simulink model "KC200GT"  (R2023a)
settings: Solver=ode1  StartTime=0.0  StopTime=1  FixedStep=1e-4  RelTol=1e-3
libraries: simulink x1
settings Model: Creator=Solal  LastModifiedBy=Solal

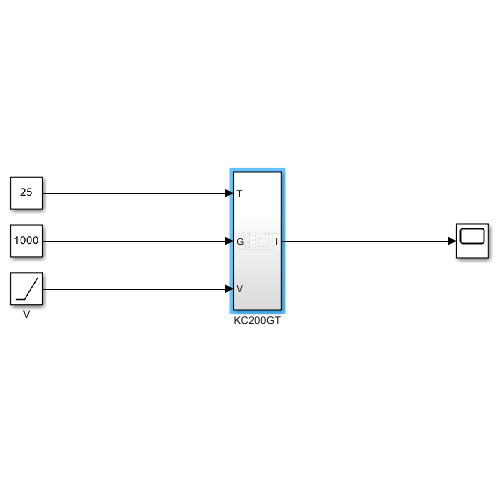
[thumbnail: Simulink's stored preview of the top-level diagram]
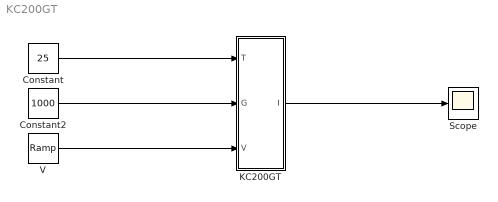
== system KC200GT ==
  Constant : Constant  Value=25
  Constant2 : Constant  Value=1000
  KC200GT : Subsystem
  Scope : Scope
  V : simulink/Sources/Ramp  slope=40  start=0  InitialOutput=0
  wires:
  Constant/1 -> KC200GT/1(T)
  Constant2/1 -> KC200GT/2(G)
  V/1 -> KC200GT/3(V)
  KC200GT/1(I) -> Scope/1

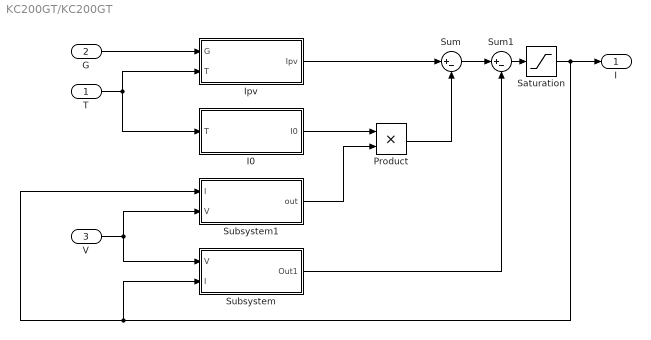
== system KC200GT/KC200GT ==
  T : Inport
  G : Inport  Port=2
  V : Inport  Port=3
  I0 : Subsystem
  Ipv : Subsystem
  Product : Product
  Saturation : Saturate  UpperLimit=inf  LowerLimit=0
  Subsystem : Subsystem
  Subsystem1 : Subsystem
  Sum : Sum  Inputs=|+-
  Sum1 : Sum  Inputs=|+-
  I : Outport
  wires:
  Ipv/1(Ipv) -> Sum/1
  I0/1(I0) -> Product/1
  Saturation/1 -> Subsystem1/1(I), Subsystem/2(I), I/1
  G/1 -> Ipv/1(G)
  Sum/1 -> Sum1/1
  T/1 -> I0/1(T), Ipv/2(T)
  V/1 -> Subsystem/1(V), Subsystem1/2(V)
  Subsystem/1(Out1) -> Sum1/2
  Subsystem1/1(out) -> Product/2
  Product/1 -> Sum/2
  Sum1/1 -> Saturation/1

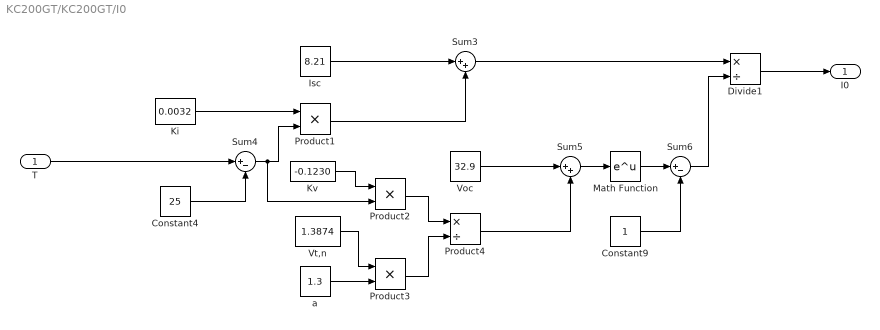
== system KC200GT/KC200GT/I0 ==
  T : Inport
  Constant4 : Constant  Value=25
  Constant9 : Constant
  Divide1 : Product  Inputs=*/
  Isc : Constant  Value=8.21
  Ki : Constant  Value=0.0032
  Kv : Constant  Value=-0.1230
  Math Function : Math
  Product1 : Product
  Product2 : Product
  Product3 : Product
  Product4 : Product  Inputs=*/
  Sum3 : Sum  Inputs=|++
  Sum4 : Sum  Inputs=|+-
  Sum5 : Sum  Inputs=|++
  Sum6 : Sum  Inputs=|+-
  Voc : Constant  Value=32.9
  Vt,n : Constant  Value=1.3874
  a : Constant  Value=1.3
  I0 : Outport
  wires:
  Sum3/1 -> Divide1/1
  Constant9/1 -> Sum6/2
  Product1/1 -> Sum3/2
  Ki/1 -> Product1/1
  Product4/1 -> Sum5/2
  Sum4/1 -> Product2/2, Product1/2
  Sum6/1 -> Divide1/2
  Math Function/1 -> Sum6/1
  Isc/1 -> Sum3/1
  Constant4/1 -> Sum4/2
  Voc/1 -> Sum5/1
  Product3/1 -> Product4/2
  Vt,n/1 -> Product3/1
  Product2/1 -> Product4/1
  a/1 -> Product3/2
  Kv/1 -> Product2/1
  T/1 -> Sum4/1
  Sum5/1 -> Math Function/1
  Divide1/1 -> I0/1

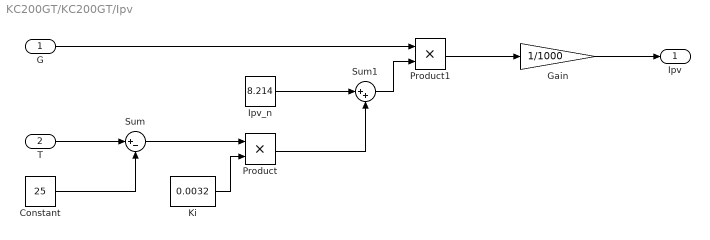
== system KC200GT/KC200GT/Ipv ==
  G : Inport
  T : Inport  Port=2
  Constant : Constant  Value=25
  Gain : Gain  Gain=1/1000
  Ipv_n : Constant  Value=8.214
  Ki : Constant  Value=0.0032
  Product : Product
  Product1 : Product
  Sum : Sum  Inputs=|+-
  Sum1 : Sum  Inputs=|++
  Ipv : Outport
  wires:
  Product/1 -> Sum1/2
  Constant/1 -> Sum/2
  Product1/1 -> Gain/1
  G/1 -> Product1/1
  Ki/1 -> Product/2
  T/1 -> Sum/1
  Ipv_n/1 -> Sum1/1
  Sum/1 -> Product/1
  Sum1/1 -> Product1/2
  Gain/1 -> Ipv/1

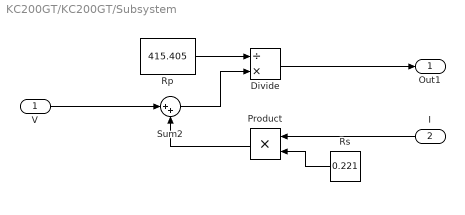
== system KC200GT/KC200GT/Subsystem ==
  V : Inport
  I : Inport  Port=2
  Divide : Product  Inputs=/*
  Product : Product
  Rp : Constant  Value=415.405
  Rs : Constant  Value=0.221
  Sum2 : Sum  Inputs=|++
  Out1 : Outport
  wires:
  I/1 -> Product/1
  V/1 -> Sum2/1
  Rs/1 -> Product/2
  Divide/1 -> Out1/1
  Rp/1 -> Divide/1
  Product/1 -> Sum2/2
  Sum2/1 -> Divide/2

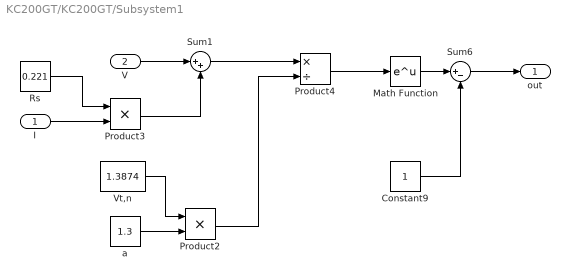
== system KC200GT/KC200GT/Subsystem1 ==
  I : Inport
  V : Inport  Port=2
  Constant9 : Constant
  Math Function : Math
  Product2 : Product
  Product3 : Product
  Product4 : Product  Inputs=*/
  Rs : Constant  Value=0.221
  Sum1 : Sum  Inputs=|++
  Sum6 : Sum  Inputs=|+-
  Vt,n : Constant  Value=1.3874
  a : Constant  Value=1.3
  out : Outport
  wires:
  I/1 -> Product3/2
  Sum6/1 -> out/1
  a/1 -> Product2/2
  Constant9/1 -> Sum6/2
  Rs/1 -> Product3/1
  Math Function/1 -> Sum6/1
  Vt,n/1 -> Product2/1
  Product2/1 -> Product4/2
  Sum1/1 -> Product4/1
  Product3/1 -> Sum1/2
  V/1 -> Sum1/1
  Product4/1 -> Math Function/1
